simulink model "perturbation_precision"  (R2024b)
settings: Solver=VariableStepAuto  StartTime=0.0  StopTime=30  MaxStep=0.1  RelTol=1e-3
settings Model: Creator=filipe  LastModifiedBy=filipe

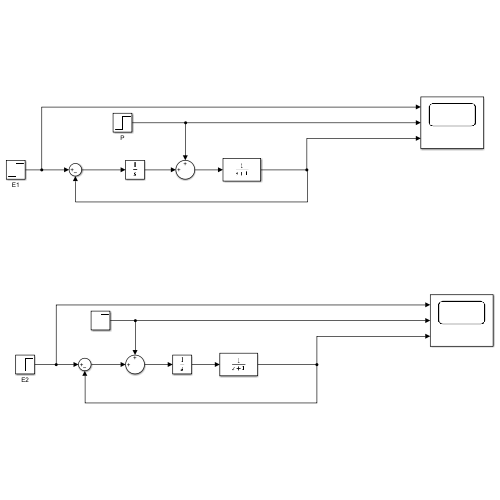
[thumbnail: Simulink's stored preview of the top-level diagram]
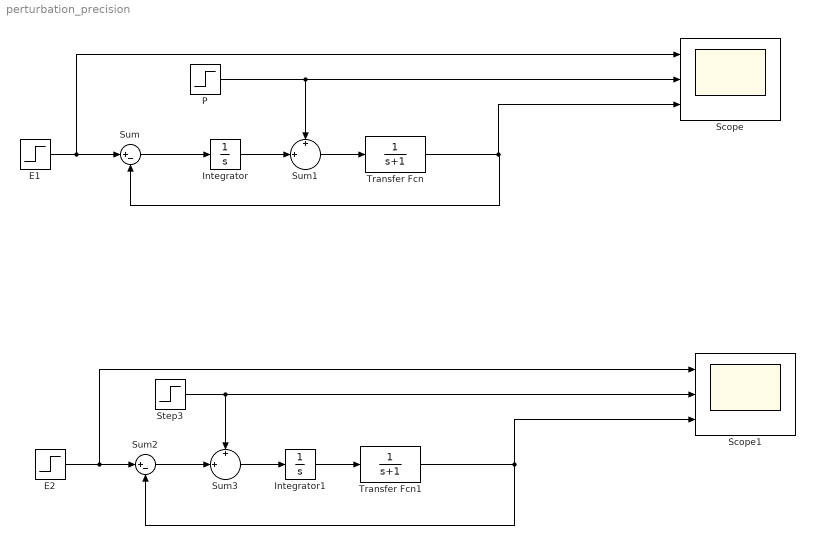
== system perturbation_precision ==
  E1 : Step  SampleTime=0
  E2 : Step  SampleTime=0
  Integrator : Integrator
  Integrator1 : Integrator
  P : Step  Time=15  After=0.5  SampleTime=0
  Scope : Scope  NumInputPorts=3
  Scope1 : Scope  NumInputPorts=3
  Step3 : Step  Time=15  After=0.5  SampleTime=0
  Sum : Sum  Inputs=|+-
  Sum1 : Sum  Inputs=+|+||
  Sum2 : Sum  Inputs=|+-
  Sum3 : Sum  Inputs=+|+||
  Transfer Fcn : TransferFcn  Denominator=[1 1]
  Transfer Fcn1 : TransferFcn  Denominator=[1 1]
  wires:
  E1/1 -> Scope/1, Sum/1
  Sum/1 -> Integrator/1
  Sum1/1 -> Transfer Fcn/1
  Transfer Fcn/1 -> Scope/3, Sum/2
  Transfer Fcn1/1 -> Sum2/2, Scope1/3
  E2/1 -> Scope1/1, Sum2/1
  Sum3/1 -> Integrator1/1
  Integrator1/1 -> Transfer Fcn1/1
  Integrator/1 -> Sum1/2
  P/1 -> Scope/2, Sum1/1
  Step3/1 -> Scope1/2, Sum3/1
  Sum2/1 -> Sum3/2
